simulink model "SHEMS_Model"  (R2025a)
settings: Solver=ode45  StartTime=0.0  StopTime=24  RelTol=1e-3
values from neighbouring files (symbols this model uses):
  E_batt_nom = 10.0    (= 10)    [shems_parameters.m]
  P_load = u(2)    [hems_controller_fcn.m]    (also in shems_parameters.m = zeros(1, N))
  P_pv = u(1)    [hems_controller_fcn.m]    (also in shems_parameters.m = (irradiance / G_peak) * P_pv_rated * eta_inverter)
  SOC_init = 50.0    (= 50)    [shems_parameters.m]
  SOC_max = 95.0    (= 95)    [hems_controller_fcn.m]    (also in shems_parameters.m)
  SOC_min = 20.0    (= 20)    [hems_controller_fcn.m]    (also in shems_parameters.m)
  time = 0:dt:24    [shems_parameters.m]
settings Model: Creator=ardhy  LastModifiedBy=ardhy
settings SolverCC: SolverResetMethod=Robust

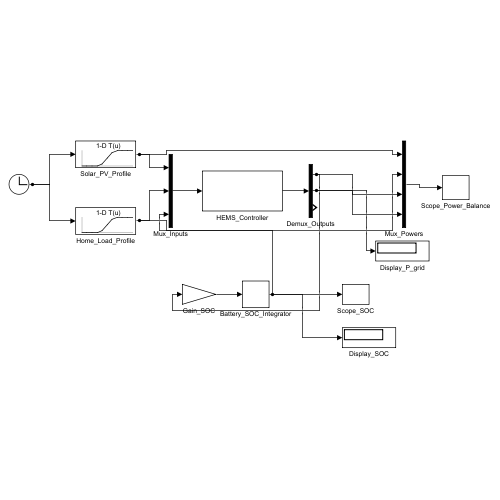
[thumbnail: Simulink's stored preview of the top-level diagram]
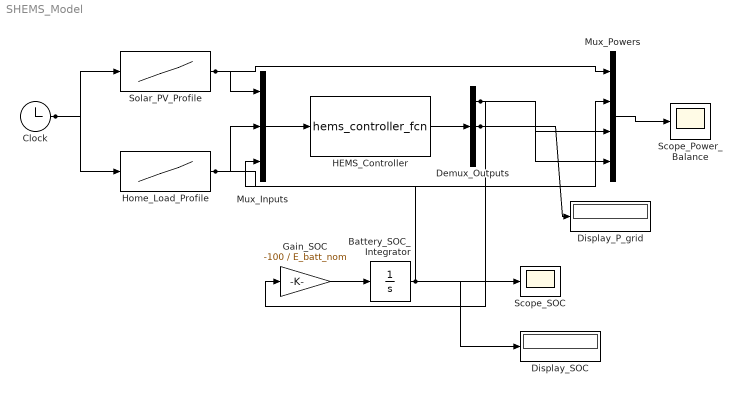
== system SHEMS_Model ==
  Battery_SOC_Integrator : Integrator  InitialCondition=SOC_init  LimitOutput=on  UpperSaturationLimit=SOC_max  LowerSaturationLimit=SOC_min
  Clock : Clock
  Demux_Outputs : Demux  Outputs=3
  Display_P_grid : Display
  Display_SOC : Display
  Gain_SOC : Gain  Gain=-100 / E_batt_nom
  HEMS_Controller : MATLABFcn  MATLABFcn=hems_controller_fcn
  Home_Load_Profile : Lookup_n-D  NumberOfTableDimensions=1  BreakpointsForDimension1=time  Table=P_load  InternalRulePriority=Speed  RndMeth=Simplest
  Mux_Inputs : Mux  Inputs=3
  Mux_Powers : Mux
  Scope_Power_Balance : Scope
  Scope_SOC : Scope
  Solar_PV_Profile : Lookup_n-D  NumberOfTableDimensions=1  BreakpointsForDimension1=time  Table=P_pv  InternalRulePriority=Speed  RndMeth=Simplest
  wires:
  Clock/1 -> Solar_PV_Profile/1, Home_Load_Profile/1
  Solar_PV_Profile/1 -> Mux_Inputs/1, Mux_Powers/1
  Home_Load_Profile/1 -> Mux_Inputs/2, Mux_Powers/2
  Battery_SOC_Integrator/1 -> Mux_Inputs/3, Scope_SOC/1, Display_SOC/1
  Mux_Inputs/1 -> HEMS_Controller/1
  HEMS_Controller/1 -> Demux_Outputs/1
  Demux_Outputs/1 -> Gain_SOC/1, Mux_Powers/3
  Gain_SOC/1 -> Battery_SOC_Integrator/1
  Demux_Outputs/2 -> Display_P_grid/1, Mux_Powers/4
  Mux_Powers/1 -> Scope_Power_Balance/1
